simulink model "asbCubeSatArchModel"  (R2025b)
settings: configuration reference "CubeSatConfigSet" (kept outside this file)
InitFcn:
  | detectChangeOrbitalElements;
settings Model: DataDictionary=asbCubeSatArchInterfaceData.sldd  Creator=The MathWorks, Inc.  LastModifiedBy=The MathWorks, Inc.
settings ConfigSetRef: SourceName=CubeSatConfigSet

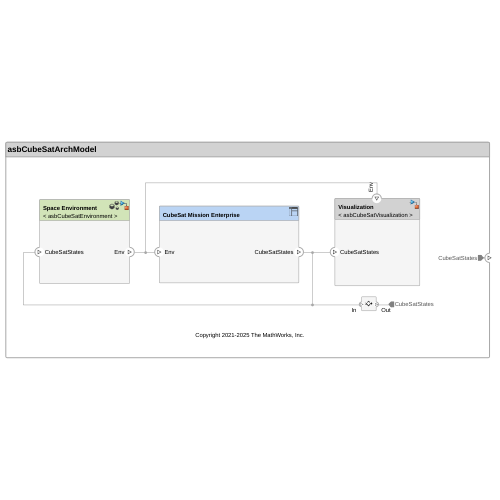
[thumbnail: Simulink's stored preview of the top-level diagram]
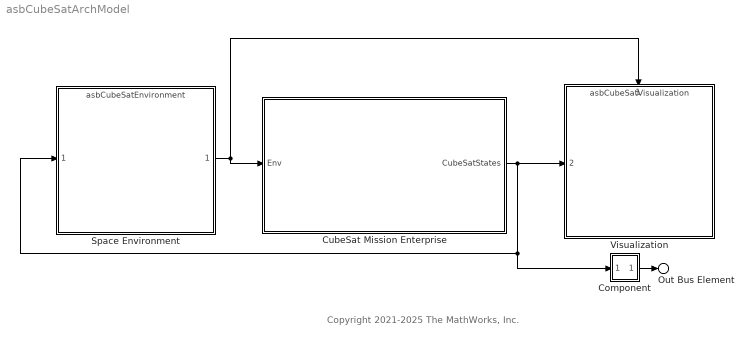
== system asbCubeSatArchModel ==
  note: Copyright 2021-2025 The MathWorks, Inc.
  Component : Subsystem
      settings: PortSchema="{\"entries\":[{\"content\":{\"margin\":10,\"minimumSpacing\":15,\"sides\":[{\"content\":{\"connectorIds\":[\"In1\"]},\"type\":\"ConnectorPlacement.EquallySpacedRectSide\",\"uuid\":\"9886ff7d-e976-4db1-93a5-6c4881d35d20\"},{\"content\":{\"connectorIds\":[\"Out1\"],\"side\":\"RIGHT\"},\"type\":\"ConnectorPlacement.EquallySpacedRectSide\",\"uuid\":\"ddfda7ac-6297-4455-a293-3eb8c5cedc24\"},{\"content\":{\"connectorIds\":[],\"side\":\"TOP\"},\"type\":\"ConnectorPlacement.EquallySpacedRectSide\",\"uuid\":\"53df18f4-c3f2-41e9-b086-6e9f9df8353a\"}]},\"type\":\"ConnectorPlacement.EquallySpacedConnector\",\"uuid\":\"ec2e31ee-cd1e-423f-b63c-a0e50b4897cf\"}],\"packageUris\":[\"http://schema.mathworks.com/mf0/Connector/R2020b\"],\"version\":\"1.0\"}"
  CubeSat Mission Enterprise : Subsystem  RequirementInfo="{}  %GIDa_b28b2482_6772_472c_87a3_7f97e1661d65"
      settings: PortSchema="{\"entries\":[{\"content\":{\"headerSize\":26,\"margin\":15,\"minimumSpacing\":25,\"sides\":[{\"content\":{\"connectorIds\":[\"In1\"]},\"type\":\"ConnectorPlacement.EquallySpacedRectSide\",\"uuid\":\"9b45e59d-ccd6-4576-99ba-beb2b78ee3b5\"},{\"content\":{\"connectorIds\":[\"Out1\"],\"side\":\"RIGHT\"},\"type\":\"ConnectorPlacement.EquallySpacedRectSide\",\"uuid\":\"e86d53dc-9e16-4af5-b392-fbf304437072\"},{\"content\":{\"connectorIds\":[],\"side\":\"TOP\"},\"type\":\"ConnectorPlacement.EquallySpacedRectSide\",\"uuid\":\"edfd08ba-6cd1-4548-8657-f8bd2c19a2e8\"}]},\"type\":\"ConnectorPlacement.EquallySpacedConnector\",\"uuid\":\"6ec86e3f-e232-4d2b-9702-b7c5151da82d\"}],\"packageUris\":[\"http://schema.mathworks.com/mf0/Connector/R2020b\"],\"version\":\"1.0\"}"
  Space Environment : ModelReference  ModelNameDialog=asbCubeSatEnvironment.slx  SimulationMode=Normal  ModelReferenceVersion=10.1
      settings: PortSchema="{\"entries\":[{\"content\":{\"headerSize\":38,\"margin\":15,\"minimumSpacing\":25,\"sides\":[{\"content\":{\"connectorIds\":[\"In1\"]},\"type\":\"ConnectorPlacement.EquallySpacedRectSide\",\"uuid\":\"f3e38669-0fba-438a-830e-4ecb3c477208\"},{\"content\":{\"connectorIds\":[\"Out1\"],\"side\":\"RIGHT\"},\"type\":\"ConnectorPlacement.EquallySpacedRectSide\",\"uuid\":\"56bbb7a2-868c-414d-930b-0bd7cd2045f0\"},{\"content\":{\"connectorIds\":[],\"side\":\"TOP\"},\"type\":\"ConnectorPlacement.EquallySpacedRectSide\",\"uuid\":\"88870cdb-fdfd-417b-9994-916f0d4ae524\"}]},\"type\":\"ConnectorPlacement.EquallySpacedConnector\",\"uuid\":\"741cde9d-e7e9-40ac-ba7b-7a3de3d6b210\"}],\"packageUris\":[\"http://schema.mathworks.com/mf0/Connector/19700101\"],\"version\":\"1.0\"}"
  Visualization : ModelReference  ModelNameDialog=asbCubeSatVisualization  SimulationMode=Normal  ModelReferenceVersion=11.7
      settings: PortSchema="{\"entries\":[{\"content\":{\"headerSize\":38,\"margin\":15,\"minimumSpacing\":25,\"sides\":[{\"content\":{\"connectorIds\":[\"In2\"]},\"type\":\"ConnectorPlacement.EquallySpacedRectSide\",\"uuid\":\"11899bdf-e452-4ab3-837e-0cb9b9384128\"},{\"content\":{\"connectorIds\":[],\"side\":\"RIGHT\"},\"type\":\"ConnectorPlacement.EquallySpacedRectSide\",\"uuid\":\"e13bda72-6c98-45bd-b419-0150b74f0acb\"},{\"content\":{\"connectorIds\":[\"In1\"],\"side\":\"TOP\"},\"type\":\"ConnectorPlacement.EquallySpacedRectSide\",\"uuid\":\"557a35da-b63d-4ba5-9926-82fbb2616f97\"}]},\"type\":\"ConnectorPlacement.EquallySpacedConnector\",\"uuid\":\"5fda5664-0755-42bb-a997-eaa89ad1d59d\"}],\"packageUris\":[\"http://schema.mathworks.com/mf0/Connector/R2020b\"],\"version\":\"1.0\"}"
  Out Bus Element : Outport  PortName=CubeSatStates
  wires:
  Space Environment/1 -> Visualization/1, CubeSat Mission Enterprise/1(Env)
  CubeSat Mission Enterprise/1(CubeSatStates) -> Component/1(In), Space Environment/1, Visualization/2
  Component/1(Out) -> Out Bus Element/1

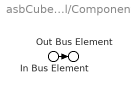
== system asbCubeSatArchModel/Component ==
  In Bus Element : Inport  PortName=In
  Out Bus Element : Outport  PortName=Out
  wires:
  In Bus Element/1 -> Out Bus Element/1

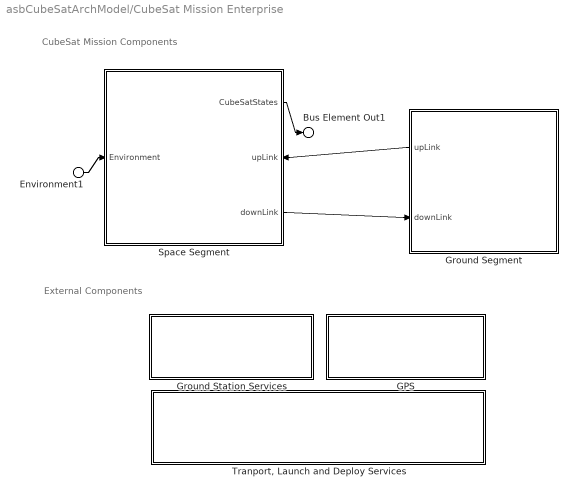
== system asbCubeSatArchModel/CubeSat Mission Enterprise ==
  note: CubeSat Mission Components
  note: External Components
  Environment1 : Inport  PortName=Env
  GPS : Subsystem
      settings: PortSchema="{\"entries\":[{\"content\":{\"headerSize\":26,\"margin\":15,\"minimumSpacing\":25,\"sides\":[{\"content\":{\"connectorIds\":[]},\"type\":\"ConnectorPlacement.EquallySpacedRectSide\",\"uuid\":\"9b45e59d-ccd6-4576-99ba-beb2b78ee3b5\"},{\"content\":{\"connectorIds\":[],\"side\":\"RIGHT\"},\"type\":\"ConnectorPlacement.EquallySpacedRectSide\",\"uuid\":\"e86d53dc-9e16-4af5-b392-fbf304437072\"},{\"content\":{\"connectorIds\":[],\"side\":\"TOP\"},\"type\":\"ConnectorPlacement.EquallySpacedRectSide\",\"uuid\":\"edfd08ba-6cd1-4548-8657-f8bd2c19a2e8\"}]},\"type\":\"ConnectorPlacement.EquallySpacedConnector\",\"uuid\":\"6ec86e3f-e232-4d2b-9702-b7c5151da82d\"}],\"packageUris\":[\"http://schema.mathworks.com/mf0/Connector/19700101\"],\"version\":\"1.0\"}"
  Ground Segment : Subsystem  RequirementInfo="{}  %GIDa_b06ae174_6660_44fc_ae78_7625ee106db0"
      settings: PortSchema="{\"entries\":[{\"content\":{\"headerSize\":26,\"margin\":15,\"minimumSpacing\":25,\"sides\":[{\"content\":{\"connectorIds\":[\"Out1\",\"In1\"]},\"type\":\"ConnectorPlacement.EquallySpacedRectSide\",\"uuid\":\"9b45e59d-ccd6-4576-99ba-beb2b78ee3b5\"},{\"content\":{\"connectorIds\":[],\"side\":\"RIGHT\"},\"type\":\"ConnectorPlacement.EquallySpacedRectSide\",\"uuid\":\"e86d53dc-9e16-4af5-b392-fbf304437072\"},{\"content\":{\"connectorIds\":[],\"side\":\"TOP\"},\"type\":\"ConnectorPlacement.EquallySpacedRectSide\",\"uuid\":\"edfd08ba-6cd1-4548-8657-f8bd2c19a2e8\"}]},\"type\":\"ConnectorPlacement.EquallySpacedConnector\",\"uuid\":\"6ec86e3f-e232-4d2b-9702-b7c5151da82d\"}],\"packageUris\":[\"http://schema.mathworks.com/mf0/Connector/19700101\"],\"version\":\"1.0\"}"
  Ground Station Services : Subsystem
      settings: PortSchema="{\"entries\":[{\"content\":{\"headerSize\":26,\"margin\":15,\"minimumSpacing\":25,\"sides\":[{\"content\":{\"connectorIds\":[]},\"type\":\"ConnectorPlacement.EquallySpacedRectSide\",\"uuid\":\"9b45e59d-ccd6-4576-99ba-beb2b78ee3b5\"},{\"content\":{\"connectorIds\":[],\"side\":\"RIGHT\"},\"type\":\"ConnectorPlacement.EquallySpacedRectSide\",\"uuid\":\"e86d53dc-9e16-4af5-b392-fbf304437072\"},{\"content\":{\"connectorIds\":[],\"side\":\"TOP\"},\"type\":\"ConnectorPlacement.EquallySpacedRectSide\",\"uuid\":\"edfd08ba-6cd1-4548-8657-f8bd2c19a2e8\"}]},\"type\":\"ConnectorPlacement.EquallySpacedConnector\",\"uuid\":\"6ec86e3f-e232-4d2b-9702-b7c5151da82d\"}],\"packageUris\":[\"http://schema.mathworks.com/mf0/Connector/19700101\"],\"version\":\"1.0\"}"
  Space Segment : Subsystem  RequirementInfo="{}  %GIDa_d5559e4d_919a_44dc_b881_614a5dae06b6"
      settings: PortSchema="{\"entries\":[{\"content\":{\"headerSize\":26,\"margin\":15,\"minimumSpacing\":25,\"sides\":[{\"content\":{\"connectorIds\":[\"In2\"]},\"type\":\"ConnectorPlacement.EquallySpacedRectSide\",\"uuid\":\"9b45e59d-ccd6-4576-99ba-beb2b78ee3b5\"},{\"content\":{\"connectorIds\":[\"Out1\",\"In1\",\"Out2\"],\"side\":\"RIGHT\"},\"type\":\"ConnectorPlacement.EquallySpacedRectSide\",\"uuid\":\"e86d53dc-9e16-4af5-b392-fbf304437072\"},{\"content\":{\"connectorIds\":[],\"side\":\"TOP\"},\"type\":\"ConnectorPlacement.EquallySpacedRectSide\",\"uuid\":\"edfd08ba-6cd1-4548-8657-f8bd2c19a2e8\"}]},\"type\":\"ConnectorPlacement.EquallySpacedConnector\",\"uuid\":\"6ec86e3f-e232-4d2b-9702-b7c5151da82d\"}],\"packageUris\":[\"http://schema.mathworks.com/mf0/Connector/R2020b\"],\"version\":\"1.0\"}"
  "Tranport, Launch and Deploy Services" : Subsystem
      settings: PortSchema="{\"entries\":[{\"content\":{\"headerSize\":26,\"margin\":15,\"minimumSpacing\":25,\"sides\":[{\"content\":{\"connectorIds\":[]},\"type\":\"ConnectorPlacement.EquallySpacedRectSide\",\"uuid\":\"9b45e59d-ccd6-4576-99ba-beb2b78ee3b5\"},{\"content\":{\"connectorIds\":[],\"side\":\"RIGHT\"},\"type\":\"ConnectorPlacement.EquallySpacedRectSide\",\"uuid\":\"e86d53dc-9e16-4af5-b392-fbf304437072\"},{\"content\":{\"connectorIds\":[],\"side\":\"TOP\"},\"type\":\"ConnectorPlacement.EquallySpacedRectSide\",\"uuid\":\"edfd08ba-6cd1-4548-8657-f8bd2c19a2e8\"}]},\"type\":\"ConnectorPlacement.EquallySpacedConnector\",\"uuid\":\"6ec86e3f-e232-4d2b-9702-b7c5151da82d\"}],\"packageUris\":[\"http://schema.mathworks.com/mf0/Connector/19700101\"],\"version\":\"1.0\"}"
  Bus Element Out1 : Outport  PortName=CubeSatStates
  wires:
  Environment1/1 -> Space Segment/2(Environment)
  Ground Segment/1(upLink) -> Space Segment/1(upLink)
  Space Segment/2(downLink) -> Ground Segment/1(downLink)
  Space Segment/1(CubeSatStates) -> Bus Element Out1/1

== system asbCubeSatArchModel/CubeSat Mission Enterprise/GPS ==

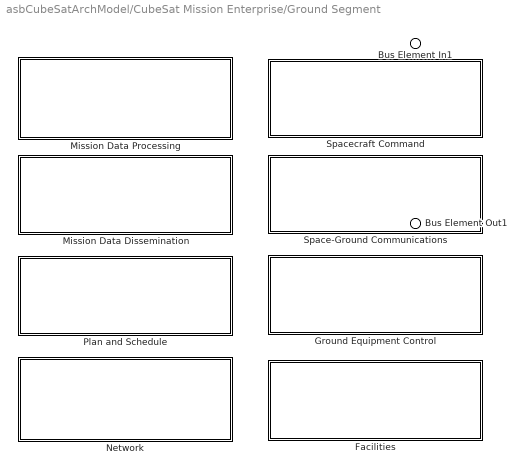
== system asbCubeSatArchModel/CubeSat Mission Enterprise/Ground Segment ==
  Bus Element In1 : Inport  PortName=downLink
  Facilities : Subsystem
      settings: PortSchema="{\"entries\":[{\"content\":{\"headerSize\":26,\"margin\":15,\"minimumSpacing\":25,\"sides\":[{\"content\":{\"connectorIds\":[]},\"type\":\"ConnectorPlacement.EquallySpacedRectSide\",\"uuid\":\"ec0b20de-43af-4595-9773-1ccab80dcb2a\"},{\"content\":{\"connectorIds\":[],\"side\":\"RIGHT\"},\"type\":\"ConnectorPlacement.EquallySpacedRectSide\",\"uuid\":\"ac6e6885-e3fb-4062-8a30-0baee43cecf2\"},{\"content\":{\"connectorIds\":[],\"side\":\"TOP\"},\"type\":\"ConnectorPlacement.EquallySpacedRectSide\",\"uuid\":\"2a1a79cc-6d5a-466f-8cc8-4618e952e6e8\"}]},\"type\":\"ConnectorPlacement.EquallySpacedConnector\",\"uuid\":\"4eb0413c-b7e8-4869-aa38-85b4ce7d1395\"}],\"packageUris\":[\"http://schema.mathworks.com/mf0/Connector/R2020b\"],\"version\":\"1.0\"}"
  Ground Equipment Control : Subsystem
      settings: PortSchema="{\"entries\":[{\"content\":{\"headerSize\":26,\"margin\":15,\"minimumSpacing\":25,\"sides\":[{\"content\":{\"connectorIds\":[]},\"type\":\"ConnectorPlacement.EquallySpacedRectSide\",\"uuid\":\"9b45e59d-ccd6-4576-99ba-beb2b78ee3b5\"},{\"content\":{\"connectorIds\":[],\"side\":\"RIGHT\"},\"type\":\"ConnectorPlacement.EquallySpacedRectSide\",\"uuid\":\"e86d53dc-9e16-4af5-b392-fbf304437072\"},{\"content\":{\"connectorIds\":[],\"side\":\"TOP\"},\"type\":\"ConnectorPlacement.EquallySpacedRectSide\",\"uuid\":\"edfd08ba-6cd1-4548-8657-f8bd2c19a2e8\"}]},\"type\":\"ConnectorPlacement.EquallySpacedConnector\",\"uuid\":\"6ec86e3f-e232-4d2b-9702-b7c5151da82d\"}],\"packageUris\":[\"http://schema.mathworks.com/mf0/Connector/19700101\"],\"version\":\"1.0\"}"
  Mission Data Dissemination : Subsystem
      settings: PortSchema="{\"entries\":[{\"content\":{\"headerSize\":26,\"margin\":15,\"minimumSpacing\":25,\"sides\":[{\"content\":{\"connectorIds\":[]},\"type\":\"ConnectorPlacement.EquallySpacedRectSide\",\"uuid\":\"9b45e59d-ccd6-4576-99ba-beb2b78ee3b5\"},{\"content\":{\"connectorIds\":[],\"side\":\"RIGHT\"},\"type\":\"ConnectorPlacement.EquallySpacedRectSide\",\"uuid\":\"e86d53dc-9e16-4af5-b392-fbf304437072\"},{\"content\":{\"connectorIds\":[],\"side\":\"TOP\"},\"type\":\"ConnectorPlacement.EquallySpacedRectSide\",\"uuid\":\"edfd08ba-6cd1-4548-8657-f8bd2c19a2e8\"}]},\"type\":\"ConnectorPlacement.EquallySpacedConnector\",\"uuid\":\"6ec86e3f-e232-4d2b-9702-b7c5151da82d\"}],\"packageUris\":[\"http://schema.mathworks.com/mf0/Connector/R2020b\"],\"version\":\"1.0\"}"
  Mission Data Processing : Subsystem
      settings: PortSchema="{\"entries\":[{\"content\":{\"headerSize\":26,\"margin\":15,\"minimumSpacing\":25,\"sides\":[{\"content\":{\"connectorIds\":[]},\"type\":\"ConnectorPlacement.EquallySpacedRectSide\",\"uuid\":\"9b45e59d-ccd6-4576-99ba-beb2b78ee3b5\"},{\"content\":{\"connectorIds\":[],\"side\":\"RIGHT\"},\"type\":\"ConnectorPlacement.EquallySpacedRectSide\",\"uuid\":\"e86d53dc-9e16-4af5-b392-fbf304437072\"},{\"content\":{\"connectorIds\":[],\"side\":\"TOP\"},\"type\":\"ConnectorPlacement.EquallySpacedRectSide\",\"uuid\":\"edfd08ba-6cd1-4548-8657-f8bd2c19a2e8\"}]},\"type\":\"ConnectorPlacement.EquallySpacedConnector\",\"uuid\":\"6ec86e3f-e232-4d2b-9702-b7c5151da82d\"}],\"packageUris\":[\"http://schema.mathworks.com/mf0/Connector/19700101\"],\"version\":\"1.0\"}"
  Network : Subsystem
      settings: PortSchema="{\"entries\":[{\"content\":{\"headerSize\":26,\"margin\":15,\"minimumSpacing\":25,\"sides\":[{\"content\":{\"connectorIds\":[]},\"type\":\"ConnectorPlacement.EquallySpacedRectSide\",\"uuid\":\"9b45e59d-ccd6-4576-99ba-beb2b78ee3b5\"},{\"content\":{\"connectorIds\":[],\"side\":\"RIGHT\"},\"type\":\"ConnectorPlacement.EquallySpacedRectSide\",\"uuid\":\"e86d53dc-9e16-4af5-b392-fbf304437072\"},{\"content\":{\"connectorIds\":[],\"side\":\"TOP\"},\"type\":\"ConnectorPlacement.EquallySpacedRectSide\",\"uuid\":\"edfd08ba-6cd1-4548-8657-f8bd2c19a2e8\"}]},\"type\":\"ConnectorPlacement.EquallySpacedConnector\",\"uuid\":\"6ec86e3f-e232-4d2b-9702-b7c5151da82d\"}],\"packageUris\":[\"http://schema.mathworks.com/mf0/Connector/19700101\"],\"version\":\"1.0\"}"
  Plan and Schedule : Subsystem
      settings: PortSchema="{\"entries\":[{\"content\":{\"headerSize\":26,\"margin\":15,\"minimumSpacing\":25,\"sides\":[{\"content\":{\"connectorIds\":[]},\"type\":\"ConnectorPlacement.EquallySpacedRectSide\",\"uuid\":\"9b45e59d-ccd6-4576-99ba-beb2b78ee3b5\"},{\"content\":{\"connectorIds\":[],\"side\":\"RIGHT\"},\"type\":\"ConnectorPlacement.EquallySpacedRectSide\",\"uuid\":\"e86d53dc-9e16-4af5-b392-fbf304437072\"},{\"content\":{\"connectorIds\":[],\"side\":\"TOP\"},\"type\":\"ConnectorPlacement.EquallySpacedRectSide\",\"uuid\":\"edfd08ba-6cd1-4548-8657-f8bd2c19a2e8\"}]},\"type\":\"ConnectorPlacement.EquallySpacedConnector\",\"uuid\":\"6ec86e3f-e232-4d2b-9702-b7c5151da82d\"}],\"packageUris\":[\"http://schema.mathworks.com/mf0/Connector/19700101\"],\"version\":\"1.0\"}"
  Space-Ground Communications : Subsystem
      settings: PortSchema="{\"entries\":[{\"content\":{\"headerSize\":26,\"margin\":15,\"minimumSpacing\":25,\"sides\":[{\"content\":{\"connectorIds\":[]},\"type\":\"ConnectorPlacement.EquallySpacedRectSide\",\"uuid\":\"9b45e59d-ccd6-4576-99ba-beb2b78ee3b5\"},{\"content\":{\"connectorIds\":[],\"side\":\"RIGHT\"},\"type\":\"ConnectorPlacement.EquallySpacedRectSide\",\"uuid\":\"e86d53dc-9e16-4af5-b392-fbf304437072\"},{\"content\":{\"connectorIds\":[],\"side\":\"TOP\"},\"type\":\"ConnectorPlacement.EquallySpacedRectSide\",\"uuid\":\"edfd08ba-6cd1-4548-8657-f8bd2c19a2e8\"}]},\"type\":\"ConnectorPlacement.EquallySpacedConnector\",\"uuid\":\"6ec86e3f-e232-4d2b-9702-b7c5151da82d\"}],\"packageUris\":[\"http://schema.mathworks.com/mf0/Connector/R2020b\"],\"version\":\"1.0\"}"
  Spacecraft Command : Subsystem
      settings: PortSchema="{\"entries\":[{\"content\":{\"headerSize\":26,\"margin\":15,\"minimumSpacing\":25,\"sides\":[{\"content\":{\"connectorIds\":[]},\"type\":\"ConnectorPlacement.EquallySpacedRectSide\",\"uuid\":\"9b45e59d-ccd6-4576-99ba-beb2b78ee3b5\"},{\"content\":{\"connectorIds\":[],\"side\":\"RIGHT\"},\"type\":\"ConnectorPlacement.EquallySpacedRectSide\",\"uuid\":\"e86d53dc-9e16-4af5-b392-fbf304437072\"},{\"content\":{\"connectorIds\":[],\"side\":\"TOP\"},\"type\":\"ConnectorPlacement.EquallySpacedRectSide\",\"uuid\":\"edfd08ba-6cd1-4548-8657-f8bd2c19a2e8\"}]},\"type\":\"ConnectorPlacement.EquallySpacedConnector\",\"uuid\":\"6ec86e3f-e232-4d2b-9702-b7c5151da82d\"}],\"packageUris\":[\"http://schema.mathworks.com/mf0/Connector/R2020b\"],\"version\":\"1.0\"}"
  Bus Element Out1 : Outport  PortName=upLink

== system asbCubeSatArchModel/CubeSat Mission Enterprise/Ground Station Services ==

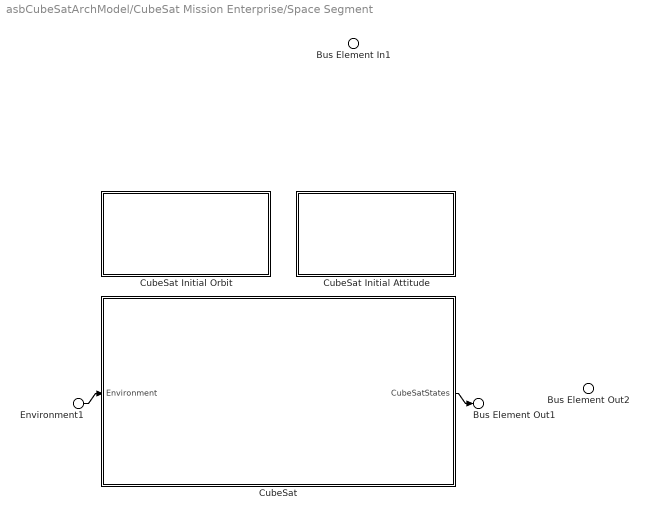
== system asbCubeSatArchModel/CubeSat Mission Enterprise/Space Segment ==
  Bus Element In1 : Inport  PortName=upLink
  Environment1 : Inport  Port=2  PortName=Environment
  CubeSat : Subsystem
      settings: PortSchema="{\"entries\":[{\"content\":{\"headerSize\":26,\"margin\":15,\"minimumSpacing\":25,\"sides\":[{\"content\":{\"connectorIds\":[\"In1\"]},\"type\":\"ConnectorPlacement.EquallySpacedRectSide\",\"uuid\":\"9b45e59d-ccd6-4576-99ba-beb2b78ee3b5\"},{\"content\":{\"connectorIds\":[\"Out1\"],\"side\":\"RIGHT\"},\"type\":\"ConnectorPlacement.EquallySpacedRectSide\",\"uuid\":\"e86d53dc-9e16-4af5-b392-fbf304437072\"},{\"content\":{\"connectorIds\":[],\"side\":\"TOP\"},\"type\":\"ConnectorPlacement.EquallySpacedRectSide\",\"uuid\":\"edfd08ba-6cd1-4548-8657-f8bd2c19a2e8\"}]},\"type\":\"ConnectorPlacement.EquallySpacedConnector\",\"uuid\":\"6ec86e3f-e232-4d2b-9702-b7c5151da82d\"}],\"packageUris\":[\"http://schema.mathworks.com/mf0/Connector/R2020b\"],\"version\":\"1.0\"}"
  CubeSat Initial Attitude : Subsystem
      settings: PortSchema="{\"entries\":[{\"content\":{\"headerSize\":26,\"margin\":15,\"minimumSpacing\":25,\"sides\":[{\"content\":{\"connectorIds\":[]},\"type\":\"ConnectorPlacement.EquallySpacedRectSide\",\"uuid\":\"9b45e59d-ccd6-4576-99ba-beb2b78ee3b5\"},{\"content\":{\"connectorIds\":[],\"side\":\"RIGHT\"},\"type\":\"ConnectorPlacement.EquallySpacedRectSide\",\"uuid\":\"e86d53dc-9e16-4af5-b392-fbf304437072\"},{\"content\":{\"connectorIds\":[],\"side\":\"TOP\"},\"type\":\"ConnectorPlacement.EquallySpacedRectSide\",\"uuid\":\"edfd08ba-6cd1-4548-8657-f8bd2c19a2e8\"}]},\"type\":\"ConnectorPlacement.EquallySpacedConnector\",\"uuid\":\"6ec86e3f-e232-4d2b-9702-b7c5151da82d\"}],\"packageUris\":[\"http://schema.mathworks.com/mf0/Connector/R2020b\"],\"version\":\"1.0\"}"
  CubeSat Initial Orbit : Subsystem  RequirementInfo="{}  %GIDa_6b67bace_5f11_42a0_bcc1_193026a664c1"
      settings: PortSchema="{\"entries\":[{\"content\":{\"headerSize\":26,\"margin\":15,\"minimumSpacing\":25,\"sides\":[{\"content\":{\"connectorIds\":[]},\"type\":\"ConnectorPlacement.EquallySpacedRectSide\",\"uuid\":\"9b45e59d-ccd6-4576-99ba-beb2b78ee3b5\"},{\"content\":{\"connectorIds\":[],\"side\":\"RIGHT\"},\"type\":\"ConnectorPlacement.EquallySpacedRectSide\",\"uuid\":\"e86d53dc-9e16-4af5-b392-fbf304437072\"},{\"content\":{\"connectorIds\":[],\"side\":\"TOP\"},\"type\":\"ConnectorPlacement.EquallySpacedRectSide\",\"uuid\":\"edfd08ba-6cd1-4548-8657-f8bd2c19a2e8\"}]},\"type\":\"ConnectorPlacement.EquallySpacedConnector\",\"uuid\":\"6ec86e3f-e232-4d2b-9702-b7c5151da82d\"}],\"packageUris\":[\"http://schema.mathworks.com/mf0/Connector/R2020b\"],\"version\":\"1.0\"}"
  Bus Element Out1 : Outport  PortName=CubeSatStates
  Bus Element Out2 : Outport  Port=2  PortName=downLink
  wires:
  Environment1/1 -> CubeSat/1(Environment)
  CubeSat/1(CubeSatStates) -> Bus Element Out1/1

== system asbCubeSatArchModel/CubeSat Mission Enterprise/Tranport, Launch and Deploy Services ==

== system asbCubeSatArchModel/CubeSat Mission Enterprise/Ground Segment/Facilities ==

== system asbCubeSatArchModel/CubeSat Mission Enterprise/Ground Segment/Ground Equipment Control ==

== system asbCubeSatArchModel/CubeSat Mission Enterprise/Ground Segment/Mission Data Dissemination ==

== system asbCubeSatArchModel/CubeSat Mission Enterprise/Ground Segment/Mission Data Processing ==

== system asbCubeSatArchModel/CubeSat Mission Enterprise/Ground Segment/Network ==

== system asbCubeSatArchModel/CubeSat Mission Enterprise/Ground Segment/Plan and Schedule ==

== system asbCubeSatArchModel/CubeSat Mission Enterprise/Ground Segment/Space-Ground Communications ==

== system asbCubeSatArchModel/CubeSat Mission Enterprise/Ground Segment/Spacecraft Command ==

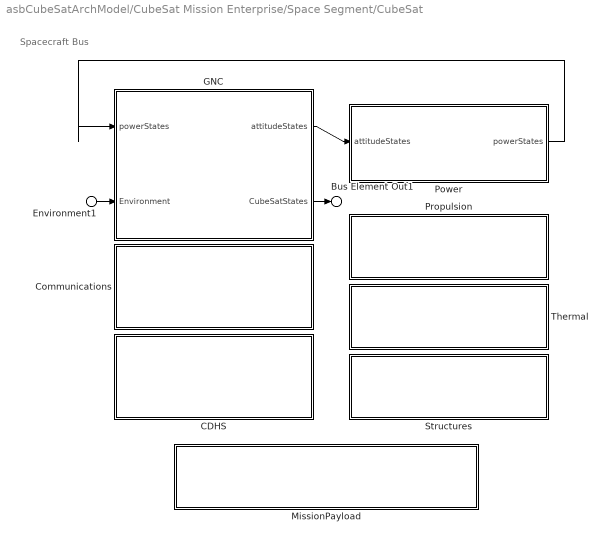
== system asbCubeSatArchModel/CubeSat Mission Enterprise/Space Segment/CubeSat ==
  note: Spacecraft Bus
  Environment1 : Inport  PortName=Environment
  CDHS : Subsystem
      settings: PortSchema="{\"entries\":[{\"content\":{\"headerSize\":26,\"margin\":15,\"minimumSpacing\":25,\"sides\":[{\"content\":{\"connectorIds\":[]},\"type\":\"ConnectorPlacement.EquallySpacedRectSide\",\"uuid\":\"9b45e59d-ccd6-4576-99ba-beb2b78ee3b5\"},{\"content\":{\"connectorIds\":[],\"side\":\"RIGHT\"},\"type\":\"ConnectorPlacement.EquallySpacedRectSide\",\"uuid\":\"e86d53dc-9e16-4af5-b392-fbf304437072\"},{\"content\":{\"connectorIds\":[],\"side\":\"TOP\"},\"type\":\"ConnectorPlacement.EquallySpacedRectSide\",\"uuid\":\"edfd08ba-6cd1-4548-8657-f8bd2c19a2e8\"}]},\"type\":\"ConnectorPlacement.EquallySpacedConnector\",\"uuid\":\"6ec86e3f-e232-4d2b-9702-b7c5151da82d\"}],\"packageUris\":[\"http://schema.mathworks.com/mf0/Connector/19700101\"],\"version\":\"1.0\"}"
  Communications : Subsystem
      settings: PortSchema="{\"entries\":[{\"content\":{\"headerSize\":26,\"margin\":15,\"minimumSpacing\":25,\"sides\":[{\"content\":{\"connectorIds\":[]},\"type\":\"ConnectorPlacement.EquallySpacedRectSide\",\"uuid\":\"9b45e59d-ccd6-4576-99ba-beb2b78ee3b5\"},{\"content\":{\"connectorIds\":[],\"side\":\"RIGHT\"},\"type\":\"ConnectorPlacement.EquallySpacedRectSide\",\"uuid\":\"e86d53dc-9e16-4af5-b392-fbf304437072\"},{\"content\":{\"connectorIds\":[],\"side\":\"TOP\"},\"type\":\"ConnectorPlacement.EquallySpacedRectSide\",\"uuid\":\"edfd08ba-6cd1-4548-8657-f8bd2c19a2e8\"}]},\"type\":\"ConnectorPlacement.EquallySpacedConnector\",\"uuid\":\"6ec86e3f-e232-4d2b-9702-b7c5151da82d\"}],\"packageUris\":[\"http://schema.mathworks.com/mf0/Connector/19700101\"],\"version\":\"1.0\"}"
  GNC : Subsystem  RequirementInfo="{}  %GIDa_dce94860_2c89_4024_b166_6039f795e48e"
      settings: PortSchema="{\"entries\":[{\"content\":{\"headerSize\":26,\"margin\":15,\"minimumSpacing\":25,\"sides\":[{\"content\":{\"connectorIds\":[\"In1\",\"In2\"]},\"type\":\"ConnectorPlacement.EquallySpacedRectSide\",\"uuid\":\"9b45e59d-ccd6-4576-99ba-beb2b78ee3b5\"},{\"content\":{\"connectorIds\":[\"Out1\",\"Out2\"],\"side\":\"RIGHT\"},\"type\":\"ConnectorPlacement.EquallySpacedRectSide\",\"uuid\":\"e86d53dc-9e16-4af5-b392-fbf304437072\"},{\"content\":{\"connectorIds\":[],\"side\":\"TOP\"},\"type\":\"ConnectorPlacement.EquallySpacedRectSide\",\"uuid\":\"edfd08ba-6cd1-4548-8657-f8bd2c19a2e8\"}]},\"type\":\"ConnectorPlacement.EquallySpacedConnector\",\"uuid\":\"6ec86e3f-e232-4d2b-9702-b7c5151da82d\"}],\"packageUris\":[\"http://schema.mathworks.com/mf0/Connector/R2020b\"],\"version\":\"1.0\"}"
  MissionPayload : Subsystem
      settings: PortSchema="{\"entries\":[{\"content\":{\"headerSize\":26,\"margin\":15,\"minimumSpacing\":25,\"sides\":[{\"content\":{\"connectorIds\":[]},\"type\":\"ConnectorPlacement.EquallySpacedRectSide\",\"uuid\":\"9b45e59d-ccd6-4576-99ba-beb2b78ee3b5\"},{\"content\":{\"connectorIds\":[],\"side\":\"RIGHT\"},\"type\":\"ConnectorPlacement.EquallySpacedRectSide\",\"uuid\":\"e86d53dc-9e16-4af5-b392-fbf304437072\"},{\"content\":{\"connectorIds\":[],\"side\":\"TOP\"},\"type\":\"ConnectorPlacement.EquallySpacedRectSide\",\"uuid\":\"edfd08ba-6cd1-4548-8657-f8bd2c19a2e8\"}]},\"type\":\"ConnectorPlacement.EquallySpacedConnector\",\"uuid\":\"6ec86e3f-e232-4d2b-9702-b7c5151da82d\"}],\"packageUris\":[\"http://schema.mathworks.com/mf0/Connector/R2020b\"],\"version\":\"1.0\"}"
  Power : Subsystem
      settings: PortSchema="{\"entries\":[{\"content\":{\"headerSize\":26,\"margin\":15,\"minimumSpacing\":25,\"sides\":[{\"content\":{\"connectorIds\":[\"In1\"]},\"type\":\"ConnectorPlacement.EquallySpacedRectSide\",\"uuid\":\"9b45e59d-ccd6-4576-99ba-beb2b78ee3b5\"},{\"content\":{\"connectorIds\":[\"Out1\"],\"side\":\"RIGHT\"},\"type\":\"ConnectorPlacement.EquallySpacedRectSide\",\"uuid\":\"e86d53dc-9e16-4af5-b392-fbf304437072\"},{\"content\":{\"connectorIds\":[],\"side\":\"TOP\"},\"type\":\"ConnectorPlacement.EquallySpacedRectSide\",\"uuid\":\"edfd08ba-6cd1-4548-8657-f8bd2c19a2e8\"}]},\"type\":\"ConnectorPlacement.EquallySpacedConnector\",\"uuid\":\"6ec86e3f-e232-4d2b-9702-b7c5151da82d\"}],\"packageUris\":[\"http://schema.mathworks.com/mf0/Connector/19700101\"],\"version\":\"1.0\"}"
  Propulsion : Subsystem
      settings: PortSchema="{\"entries\":[{\"content\":{\"headerSize\":26,\"margin\":15,\"minimumSpacing\":25,\"sides\":[{\"content\":{\"connectorIds\":[]},\"type\":\"ConnectorPlacement.EquallySpacedRectSide\",\"uuid\":\"9b45e59d-ccd6-4576-99ba-beb2b78ee3b5\"},{\"content\":{\"connectorIds\":[],\"side\":\"RIGHT\"},\"type\":\"ConnectorPlacement.EquallySpacedRectSide\",\"uuid\":\"e86d53dc-9e16-4af5-b392-fbf304437072\"},{\"content\":{\"connectorIds\":[],\"side\":\"TOP\"},\"type\":\"ConnectorPlacement.EquallySpacedRectSide\",\"uuid\":\"edfd08ba-6cd1-4548-8657-f8bd2c19a2e8\"}]},\"type\":\"ConnectorPlacement.EquallySpacedConnector\",\"uuid\":\"6ec86e3f-e232-4d2b-9702-b7c5151da82d\"}],\"packageUris\":[\"http://schema.mathworks.com/mf0/Connector/R2020b\"],\"version\":\"1.0\"}"
  Structures : Subsystem
      settings: PortSchema="{\"entries\":[{\"content\":{\"headerSize\":26,\"margin\":15,\"minimumSpacing\":25,\"sides\":[{\"content\":{\"connectorIds\":[]},\"type\":\"ConnectorPlacement.EquallySpacedRectSide\",\"uuid\":\"9b45e59d-ccd6-4576-99ba-beb2b78ee3b5\"},{\"content\":{\"connectorIds\":[],\"side\":\"RIGHT\"},\"type\":\"ConnectorPlacement.EquallySpacedRectSide\",\"uuid\":\"e86d53dc-9e16-4af5-b392-fbf304437072\"},{\"content\":{\"connectorIds\":[],\"side\":\"TOP\"},\"type\":\"ConnectorPlacement.EquallySpacedRectSide\",\"uuid\":\"edfd08ba-6cd1-4548-8657-f8bd2c19a2e8\"}]},\"type\":\"ConnectorPlacement.EquallySpacedConnector\",\"uuid\":\"6ec86e3f-e232-4d2b-9702-b7c5151da82d\"}],\"packageUris\":[\"http://schema.mathworks.com/mf0/Connector/19700101\"],\"version\":\"1.0\"}"
  Thermal : Subsystem
      settings: PortSchema="{\"entries\":[{\"content\":{\"headerSize\":26,\"margin\":15,\"minimumSpacing\":25,\"sides\":[{\"content\":{\"connectorIds\":[]},\"type\":\"ConnectorPlacement.EquallySpacedRectSide\",\"uuid\":\"9b45e59d-ccd6-4576-99ba-beb2b78ee3b5\"},{\"content\":{\"connectorIds\":[],\"side\":\"RIGHT\"},\"type\":\"ConnectorPlacement.EquallySpacedRectSide\",\"uuid\":\"e86d53dc-9e16-4af5-b392-fbf304437072\"},{\"content\":{\"connectorIds\":[],\"side\":\"TOP\"},\"type\":\"ConnectorPlacement.EquallySpacedRectSide\",\"uuid\":\"edfd08ba-6cd1-4548-8657-f8bd2c19a2e8\"}]},\"type\":\"ConnectorPlacement.EquallySpacedConnector\",\"uuid\":\"6ec86e3f-e232-4d2b-9702-b7c5151da82d\"}],\"packageUris\":[\"http://schema.mathworks.com/mf0/Connector/R2020b\"],\"version\":\"1.0\"}"
  Bus Element Out1 : Outport  PortName=CubeSatStates
  wires:
  Environment1/1 -> GNC/2(Environment)
  GNC/1(attitudeStates) -> Power/1(attitudeStates)
  Power/1(powerStates) -> GNC/1(powerStates)
  GNC/2(CubeSatStates) -> Bus Element Out1/1

== system asbCubeSatArchModel/CubeSat Mission Enterprise/Space Segment/CubeSat Initial Attitude ==
  note: Use Attitude stereotype to set initial attitude state

== system asbCubeSatArchModel/CubeSat Mission Enterprise/Space Segment/CubeSat Initial Orbit ==
  note: Use Orbit stereotype to set initial orbit state

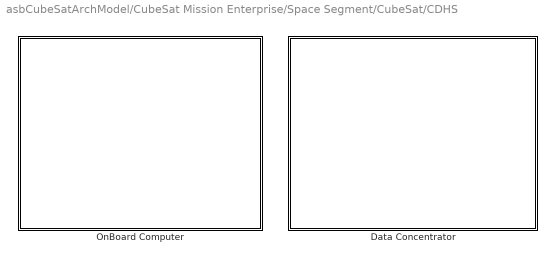
== system asbCubeSatArchModel/CubeSat Mission Enterprise/Space Segment/CubeSat/CDHS ==
  Data Concentrator : Subsystem
      settings: PortSchema="{\"entries\":[{\"content\":{\"headerSize\":26,\"margin\":15,\"minimumSpacing\":25,\"sides\":[{\"content\":{\"connectorIds\":[]},\"type\":\"ConnectorPlacement.EquallySpacedRectSide\",\"uuid\":\"5f91b340-2dca-474f-99b1-4cfb93e98d8a\"},{\"content\":{\"connectorIds\":[],\"side\":\"RIGHT\"},\"type\":\"ConnectorPlacement.EquallySpacedRectSide\",\"uuid\":\"d2e4d2f7-eaea-406c-8999-5255faa209a3\"},{\"content\":{\"connectorIds\":[],\"side\":\"TOP\"},\"type\":\"ConnectorPlacement.EquallySpacedRectSide\",\"uuid\":\"8064b484-3a4f-43f4-8560-07d3e2dea7d6\"}]},\"type\":\"ConnectorPlacement.EquallySpacedConnector\",\"uuid\":\"b547807e-0571-4405-b6f1-7ad363b80218\"}],\"packageUris\":[\"http://schema.mathworks.com/mf0/Connector/R2020b\"],\"version\":\"1.0\"}"
  OnBoard Computer : Subsystem
      settings: PortSchema="{\"entries\":[{\"content\":{\"headerSize\":26,\"margin\":15,\"minimumSpacing\":25,\"sides\":[{\"content\":{\"connectorIds\":[]},\"type\":\"ConnectorPlacement.EquallySpacedRectSide\",\"uuid\":\"5f91b340-2dca-474f-99b1-4cfb93e98d8a\"},{\"content\":{\"connectorIds\":[],\"side\":\"RIGHT\"},\"type\":\"ConnectorPlacement.EquallySpacedRectSide\",\"uuid\":\"d2e4d2f7-eaea-406c-8999-5255faa209a3\"},{\"content\":{\"connectorIds\":[],\"side\":\"TOP\"},\"type\":\"ConnectorPlacement.EquallySpacedRectSide\",\"uuid\":\"8064b484-3a4f-43f4-8560-07d3e2dea7d6\"}]},\"type\":\"ConnectorPlacement.EquallySpacedConnector\",\"uuid\":\"b547807e-0571-4405-b6f1-7ad363b80218\"}],\"packageUris\":[\"http://schema.mathworks.com/mf0/Connector/R2020b\"],\"version\":\"1.0\"}"

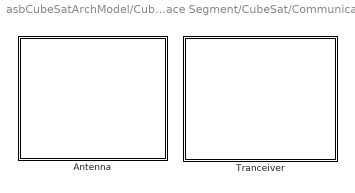
== system asbCubeSatArchModel/CubeSat Mission Enterprise/Space Segment/CubeSat/Communications ==
  Antenna : Subsystem
      settings: PortSchema="{\"entries\":[{\"content\":{\"headerSize\":26,\"margin\":15,\"minimumSpacing\":25,\"sides\":[{\"content\":{\"connectorIds\":[]},\"type\":\"ConnectorPlacement.EquallySpacedRectSide\",\"uuid\":\"5f91b340-2dca-474f-99b1-4cfb93e98d8a\"},{\"content\":{\"connectorIds\":[],\"side\":\"RIGHT\"},\"type\":\"ConnectorPlacement.EquallySpacedRectSide\",\"uuid\":\"d2e4d2f7-eaea-406c-8999-5255faa209a3\"},{\"content\":{\"connectorIds\":[],\"side\":\"TOP\"},\"type\":\"ConnectorPlacement.EquallySpacedRectSide\",\"uuid\":\"8064b484-3a4f-43f4-8560-07d3e2dea7d6\"}]},\"type\":\"ConnectorPlacement.EquallySpacedConnector\",\"uuid\":\"b547807e-0571-4405-b6f1-7ad363b80218\"}],\"packageUris\":[\"http://schema.mathworks.com/mf0/Connector/R2020b\"],\"version\":\"1.0\"}"
  Tranceiver : Subsystem
      settings: PortSchema="{\"entries\":[{\"content\":{\"headerSize\":26,\"margin\":15,\"minimumSpacing\":25,\"sides\":[{\"content\":{\"connectorIds\":[]},\"type\":\"ConnectorPlacement.EquallySpacedRectSide\",\"uuid\":\"5f91b340-2dca-474f-99b1-4cfb93e98d8a\"},{\"content\":{\"connectorIds\":[],\"side\":\"RIGHT\"},\"type\":\"ConnectorPlacement.EquallySpacedRectSide\",\"uuid\":\"d2e4d2f7-eaea-406c-8999-5255faa209a3\"},{\"content\":{\"connectorIds\":[],\"side\":\"TOP\"},\"type\":\"ConnectorPlacement.EquallySpacedRectSide\",\"uuid\":\"8064b484-3a4f-43f4-8560-07d3e2dea7d6\"}]},\"type\":\"ConnectorPlacement.EquallySpacedConnector\",\"uuid\":\"b547807e-0571-4405-b6f1-7ad363b80218\"}],\"packageUris\":[\"http://schema.mathworks.com/mf0/Connector/R2020b\"],\"version\":\"1.0\"}"

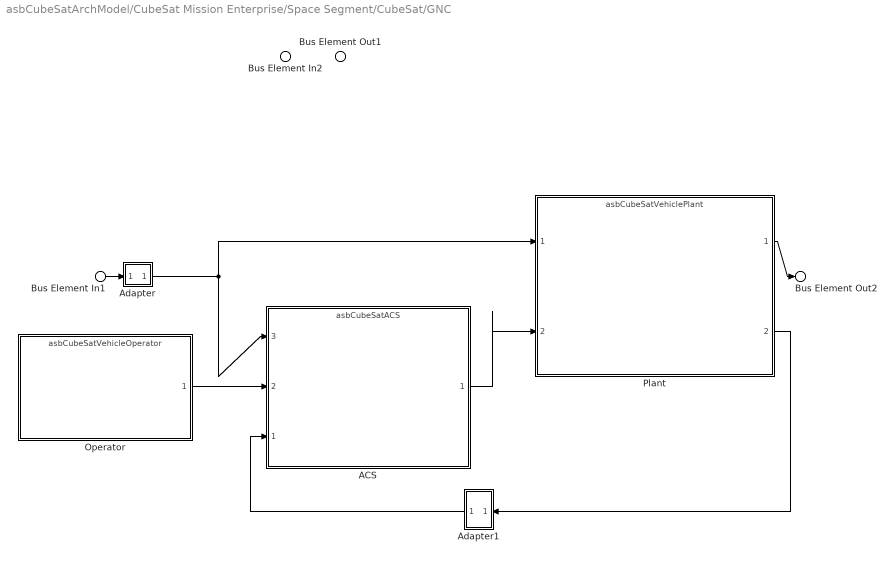
== system asbCubeSatArchModel/CubeSat Mission Enterprise/Space Segment/CubeSat/GNC ==
  Bus Element In2 : Inport  PortName=powerStates
  Bus Element In1 : Inport  Port=2  PortName=Environment
  ACS : ModelReference  ModelNameDialog=asbCubeSatACS  SimulationMode=Normal  ModelReferenceVersion=7.0
      settings: PortSchema="{\"entries\":[{\"content\":{\"headerSize\":38,\"margin\":15,\"minimumSpacing\":25,\"sides\":[{\"content\":{\"connectorIds\":[\"In3\",\"In2\",\"In1\"]},\"type\":\"ConnectorPlacement.EquallySpacedRectSide\",\"uuid\":\"0f167fc6-742e-49a6-ba84-7432b698566b\"},{\"content\":{\"connectorIds\":[\"Out1\"],\"side\":\"RIGHT\"},\"type\":\"ConnectorPlacement.EquallySpacedRectSide\",\"uuid\":\"3739c3b1-9e94-48d6-b273-772045adf57e\"},{\"content\":{\"connectorIds\":[],\"side\":\"TOP\"},\"type\":\"ConnectorPlacement.EquallySpacedRectSide\",\"uuid\":\"85e3313f-7b52-412d-a268-8976d9c4c82a\"},{\"content\":{\"connectorIds\":[],\"side\":\"HIDDEN\"},\"type\":\"ConnectorPlacement.EquallySpacedRectSide\",\"uuid\":\"31b4754e-d861-4dca-8700-99ce83c843d7\"}]},\"type\":\"ConnectorPlacement.EquallySpacedConnector\",\"uuid\":\"359d3eed-f1ba-4819-bbac-059d00dff13f\"}],\"packageUris\":[\"http://schema.mathworks.com/mf0/Connector/R2020b\"],\"version\":\"1.0\"}"
  Adapter : Subsystem
      settings: PortSchema="{\"entries\":[{\"content\":{\"margin\":10,\"minimumSpacing\":15,\"sides\":[{\"content\":{\"connectorIds\":[\"In1\"]},\"type\":\"ConnectorPlacement.EquallySpacedRectSide\",\"uuid\":\"0f167fc6-742e-49a6-ba84-7432b698566b\"},{\"content\":{\"connectorIds\":[\"Out1\"],\"side\":\"RIGHT\"},\"type\":\"ConnectorPlacement.EquallySpacedRectSide\",\"uuid\":\"3739c3b1-9e94-48d6-b273-772045adf57e\"},{\"content\":{\"connectorIds\":[],\"side\":\"TOP\"},\"type\":\"ConnectorPlacement.EquallySpacedRectSide\",\"uuid\":\"85e3313f-7b52-412d-a268-8976d9c4c82a\"},{\"content\":{\"connectorIds\":[],\"side\":\"HIDDEN\"},\"type\":\"ConnectorPlacement.EquallySpacedRectSide\",\"uuid\":\"31b4754e-d861-4dca-8700-99ce83c843d7\"}]},\"type\":\"ConnectorPlacement.EquallySpacedConnector\",\"uuid\":\"359d3eed-f1ba-4819-bbac-059d00dff13f\"}],\"packageUris\":[\"http://schema.mathworks.com/mf0/Connector/R2020b\"],\"version\":\"1.0\"}"
  Adapter1 : Subsystem
      settings: PortSchema="{\"entries\":[{\"content\":{\"margin\":10,\"minimumSpacing\":15,\"sides\":[{\"content\":{\"connectorIds\":[\"Out1\"]},\"type\":\"ConnectorPlacement.EquallySpacedRectSide\",\"uuid\":\"0f167fc6-742e-49a6-ba84-7432b698566b\"},{\"content\":{\"connectorIds\":[\"In1\"],\"side\":\"RIGHT\"},\"type\":\"ConnectorPlacement.EquallySpacedRectSide\",\"uuid\":\"3739c3b1-9e94-48d6-b273-772045adf57e\"},{\"content\":{\"connectorIds\":[],\"side\":\"TOP\"},\"type\":\"ConnectorPlacement.EquallySpacedRectSide\",\"uuid\":\"85e3313f-7b52-412d-a268-8976d9c4c82a\"},{\"content\":{\"connectorIds\":[],\"side\":\"HIDDEN\"},\"type\":\"ConnectorPlacement.EquallySpacedRectSide\",\"uuid\":\"31b4754e-d861-4dca-8700-99ce83c843d7\"}]},\"type\":\"ConnectorPlacement.EquallySpacedConnector\",\"uuid\":\"359d3eed-f1ba-4819-bbac-059d00dff13f\"}],\"packageUris\":[\"http://schema.mathworks.com/mf0/Connector/R2020b\"],\"version\":\"1.0\"}"
  Operator : ModelReference  ModelNameDialog=asbCubeSatVehicleOperator.slx  SimulationMode=Normal  ModelReferenceVersion=5.0
      settings: PortSchema="{\"entries\":[{\"content\":{\"headerSize\":38,\"margin\":15,\"minimumSpacing\":25,\"sides\":[{\"content\":{\"connectorIds\":[]},\"type\":\"ConnectorPlacement.EquallySpacedRectSide\",\"uuid\":\"0cfa3760-6acd-4ee9-b963-b5fbd04f8f00\"},{\"content\":{\"connectorIds\":[\"Out1\"],\"side\":\"RIGHT\"},\"type\":\"ConnectorPlacement.EquallySpacedRectSide\",\"uuid\":\"77ddd3d4-6692-4839-8cf9-45c7d2a217c2\"},{\"content\":{\"connectorIds\":[],\"side\":\"TOP\"},\"type\":\"ConnectorPlacement.EquallySpacedRectSide\",\"uuid\":\"8d936f89-fcb3-43a7-b6aa-fe007208be1f\"},{\"content\":{\"connectorIds\":[],\"side\":\"HIDDEN\"},\"type\":\"ConnectorPlacement.EquallySpacedRectSide\",\"uuid\":\"226e0ead-de34-4bf0-af80-010c29a26ac8\"}]},\"type\":\"ConnectorPlacement.EquallySpacedConnector\",\"uuid\":\"8760ac77-0d6c-4b36-b848-bf5fd4811ef2\"}],\"packageUris\":[\"http://schema.mathworks.com/mf0/Connector/R2020b\"],\"version\":\"1.0\"}"
  Plant : ModelReference  ModelNameDialog=asbCubeSatVehiclePlant.slx  SimulationMode=Normal  ModelReferenceVersion=6.0
      settings: PortSchema="{\"entries\":[{\"content\":{\"headerSize\":38,\"margin\":15,\"minimumSpacing\":25,\"sides\":[{\"content\":{\"connectorIds\":[\"In1\",\"In2\"]},\"type\":\"ConnectorPlacement.EquallySpacedRectSide\",\"uuid\":\"03f9f3cf-bad9-4ee2-9ea8-9738e2c4045a\"},{\"content\":{\"connectorIds\":[\"Out1\",\"Out2\"],\"side\":\"RIGHT\"},\"type\":\"ConnectorPlacement.EquallySpacedRectSide\",\"uuid\":\"a92bb464-fb2e-4a9d-9894-a6e38f24e9d5\"},{\"content\":{\"connectorIds\":[],\"side\":\"TOP\"},\"type\":\"ConnectorPlacement.EquallySpacedRectSide\",\"uuid\":\"549ebd3b-d1ab-424b-a511-2a627dad6dc4\"}]},\"type\":\"ConnectorPlacement.EquallySpacedConnector\",\"uuid\":\"0d138b15-5b32-4458-951b-b6abbba02272\"}],\"packageUris\":[\"http://schema.mathworks.com/mf0/Connector/R2020b\"],\"version\":\"1.0\"}"
  Bus Element Out1 : Outport  PortName=attitudeStates
  Bus Element Out2 : Outport  Port=2  PortName=CubeSatStates
  wires:
  Bus Element In1/1 -> Adapter/1(Environment)
  Adapter/1(Out) -> Plant/1, ACS/3
  ACS/1 -> Plant/2
  Plant/2 -> Adapter1/1(SensorsOut)
  Adapter1/1(Input) -> ACS/1
  Operator/1 -> ACS/2
  Plant/1 -> Bus Element Out2/1

== system asbCubeSatArchModel/CubeSat Mission Enterprise/Space Segment/CubeSat/MissionPayload ==

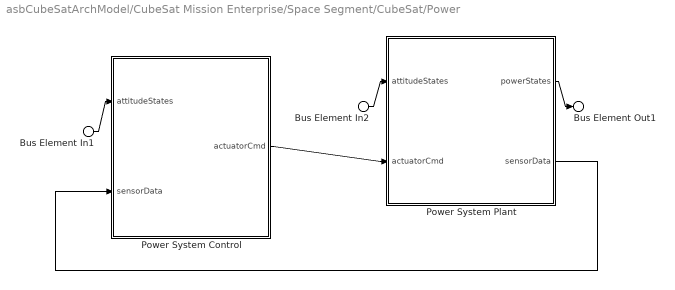
== system asbCubeSatArchModel/CubeSat Mission Enterprise/Space Segment/CubeSat/Power ==
  Bus Element In1 : Inport  PortName=attitudeStates
  Bus Element In2 : Inport  PortName=attitudeStates
  Power System Control : Subsystem  VariantControl=Choice_1
      settings: PortSchema="{\"entries\":[{\"content\":{\"headerSize\":26,\"margin\":15,\"minimumSpacing\":25,\"sides\":[{\"content\":{\"connectorIds\":[\"In1\",\"In2\"]},\"type\":\"ConnectorPlacement.EquallySpacedRectSide\",\"uuid\":\"796081c6-2161-46d9-94c7-9250e1efb39a\"},{\"content\":{\"connectorIds\":[\"Out1\"],\"side\":\"RIGHT\"},\"type\":\"ConnectorPlacement.EquallySpacedRectSide\",\"uuid\":\"b842dbfb-bf0a-4727-8e1c-eb47e2e48592\"},{\"content\":{\"connectorIds\":[],\"side\":\"TOP\"},\"type\":\"ConnectorPlacement.EquallySpacedRectSide\",\"uuid\":\"8005fa62-28e9-4165-9a4c-522b7a46ac73\"}]},\"type\":\"ConnectorPlacement.EquallySpacedConnector\",\"uuid\":\"9e1f4b76-5919-4e1e-b3b0-b0d66d2c7f29\"}],\"packageUris\":[\"http://schema.mathworks.com/mf0/Connector/R2020b\"],\"version\":\"1.0\"}"
  Power System Plant : Subsystem  VariantControl=Choice_1
      settings: PortSchema="{\"entries\":[{\"content\":{\"headerSize\":26,\"margin\":15,\"minimumSpacing\":25,\"sides\":[{\"content\":{\"connectorIds\":[\"In1\",\"In2\"]},\"type\":\"ConnectorPlacement.EquallySpacedRectSide\",\"uuid\":\"796081c6-2161-46d9-94c7-9250e1efb39a\"},{\"content\":{\"connectorIds\":[\"Out1\",\"Out2\"],\"side\":\"RIGHT\"},\"type\":\"ConnectorPlacement.EquallySpacedRectSide\",\"uuid\":\"b842dbfb-bf0a-4727-8e1c-eb47e2e48592\"},{\"content\":{\"connectorIds\":[],\"side\":\"TOP\"},\"type\":\"ConnectorPlacement.EquallySpacedRectSide\",\"uuid\":\"8005fa62-28e9-4165-9a4c-522b7a46ac73\"}]},\"type\":\"ConnectorPlacement.EquallySpacedConnector\",\"uuid\":\"9e1f4b76-5919-4e1e-b3b0-b0d66d2c7f29\"}],\"packageUris\":[\"http://schema.mathworks.com/mf0/Connector/R2020b\"],\"version\":\"1.0\"}"
  Bus Element Out1 : Outport  PortName=powerStates
  wires:
  Power System Control/1(actuatorCmd) -> Power System Plant/2(actuatorCmd)
  Power System Plant/2(sensorData) -> Power System Control/2(sensorData)
  Bus Element In1/1 -> Power System Control/1(attitudeStates)
  Power System Plant/1(powerStates) -> Bus Element Out1/1
  Bus Element In2/1 -> Power System Plant/1(attitudeStates)

== system asbCubeSatArchModel/CubeSat Mission Enterprise/Space Segment/CubeSat/Propulsion ==

== system asbCubeSatArchModel/CubeSat Mission Enterprise/Space Segment/CubeSat/Structures ==

== system asbCubeSatArchModel/CubeSat Mission Enterprise/Space Segment/CubeSat/Thermal ==

== system asbCubeSatArchModel/CubeSat Mission Enterprise/Space Segment/CubeSat/CDHS/Data Concentrator ==

== system asbCubeSatArchModel/CubeSat Mission Enterprise/Space Segment/CubeSat/CDHS/OnBoard Computer ==

== system asbCubeSatArchModel/CubeSat Mission Enterprise/Space Segment/CubeSat/Communications/Antenna ==

== system asbCubeSatArchModel/CubeSat Mission Enterprise/Space Segment/CubeSat/Communications/Tranceiver ==

== system asbCubeSatArchModel/CubeSat Mission Enterprise/Space Segment/CubeSat/GNC/Adapter ==
  In Bus Element : Inport  PortName=Environment
  Out Bus Element : Outport  PortName=Out
  wires:
  In Bus Element/1 -> Out Bus Element/1

== system asbCubeSatArchModel/CubeSat Mission Enterprise/Space Segment/CubeSat/GNC/Adapter1 ==
  In Bus Element : Inport  PortName=SensorsOut
  Out Bus Element : Outport  PortName=Input
  wires:
  In Bus Element/1 -> Out Bus Element/1

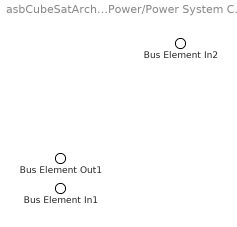
== system asbCubeSatArchModel/CubeSat Mission Enterprise/Space Segment/CubeSat/Power/Power System Control ==
  Bus Element In2 : Inport  PortName=attitudeStates
  Bus Element In1 : Inport  Port=2  PortName=sensorData
  Bus Element Out1 : Outport  PortName=actuatorCmd

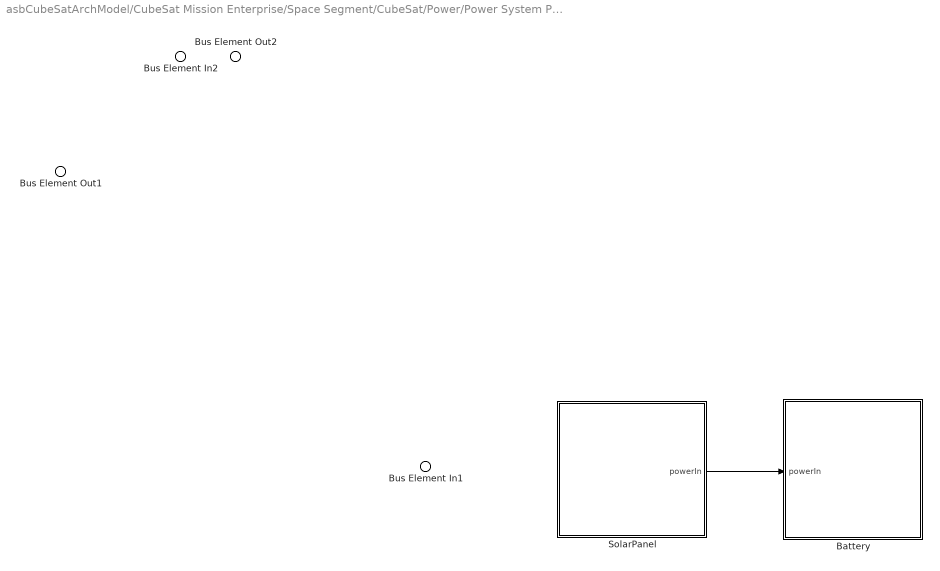
== system asbCubeSatArchModel/CubeSat Mission Enterprise/Space Segment/CubeSat/Power/Power System Plant ==
  Bus Element In2 : Inport  PortName=attitudeStates
  Bus Element In1 : Inport  Port=2  PortName=actuatorCmd
  Battery : Subsystem
      settings: PortSchema="{\"entries\":[{\"content\":{\"headerSize\":26,\"margin\":15,\"minimumSpacing\":25,\"sides\":[{\"content\":{\"connectorIds\":[\"In1\"]},\"type\":\"ConnectorPlacement.EquallySpacedRectSide\",\"uuid\":\"99007498-99ba-4c23-a0a0-87e1543943ee\"},{\"content\":{\"connectorIds\":[],\"side\":\"RIGHT\"},\"type\":\"ConnectorPlacement.EquallySpacedRectSide\",\"uuid\":\"554f3d31-4e95-4b23-9d3b-85f383ee0045\"},{\"content\":{\"connectorIds\":[],\"side\":\"TOP\"},\"type\":\"ConnectorPlacement.EquallySpacedRectSide\",\"uuid\":\"16cf11e7-d1a7-4edd-b8c5-05af2e73c5bd\"}]},\"type\":\"ConnectorPlacement.EquallySpacedConnector\",\"uuid\":\"0a651afa-d7fb-4b32-a21c-81d6f3c917ae\"}],\"packageUris\":[\"http://schema.mathworks.com/mf0/Connector/R2020b\"],\"version\":\"1.0\"}"
  SolarPanel : Subsystem  RequirementInfo="{}  %GIDa_4f725f0c_e8f4_4f8d_a212_700d35e9a783"
      settings: PortSchema="{\"entries\":[{\"content\":{\"headerSize\":26,\"margin\":15,\"minimumSpacing\":25,\"sides\":[{\"content\":{\"connectorIds\":[]},\"type\":\"ConnectorPlacement.EquallySpacedRectSide\",\"uuid\":\"bdb7f036-cfc5-488a-888f-b9d18995973e\"},{\"content\":{\"connectorIds\":[\"Out1\"],\"side\":\"RIGHT\"},\"type\":\"ConnectorPlacement.EquallySpacedRectSide\",\"uuid\":\"bf580f20-7193-4743-ad48-17eb92535429\"},{\"content\":{\"connectorIds\":[],\"side\":\"TOP\"},\"type\":\"ConnectorPlacement.EquallySpacedRectSide\",\"uuid\":\"da6f3a46-474d-4698-8115-df2cb74be4ae\"}]},\"type\":\"ConnectorPlacement.EquallySpacedConnector\",\"uuid\":\"514a736b-bd6f-43cb-ac87-4eaa6b5005de\"}],\"packageUris\":[\"http://schema.mathworks.com/mf0/Connector/R2020b\"],\"version\":\"1.0\"}"
  Bus Element Out2 : Outport  PortName=powerStates
  Bus Element Out1 : Outport  Port=2  PortName=sensorData
  wires:
  SolarPanel/1(powerIn) -> Battery/1(powerIn)

== system asbCubeSatArchModel/CubeSat Mission Enterprise/Space Segment/CubeSat/Power/Power System Plant/Battery ==
  Bus Element In1 : Inport  PortName=powerIn
  BatteryCell : Subsystem
      settings: PortSchema="{\"entries\":[{\"content\":{\"headerSize\":26,\"margin\":15,\"minimumSpacing\":25,\"sides\":[{\"content\":{\"connectorIds\":[]},\"type\":\"ConnectorPlacement.EquallySpacedRectSide\",\"uuid\":\"bdb7f036-cfc5-488a-888f-b9d18995973e\"},{\"content\":{\"connectorIds\":[],\"side\":\"RIGHT\"},\"type\":\"ConnectorPlacement.EquallySpacedRectSide\",\"uuid\":\"bf580f20-7193-4743-ad48-17eb92535429\"},{\"content\":{\"connectorIds\":[],\"side\":\"TOP\"},\"type\":\"ConnectorPlacement.EquallySpacedRectSide\",\"uuid\":\"da6f3a46-474d-4698-8115-df2cb74be4ae\"}]},\"type\":\"ConnectorPlacement.EquallySpacedConnector\",\"uuid\":\"514a736b-bd6f-43cb-ac87-4eaa6b5005de\"}],\"packageUris\":[\"http://schema.mathworks.com/mf0/Connector/19700101\"],\"version\":\"1.0\"}"

== system asbCubeSatArchModel/CubeSat Mission Enterprise/Space Segment/CubeSat/Power/Power System Plant/SolarPanel ==
  SolarPanelCell : Subsystem
      settings: PortSchema="{\"entries\":[{\"content\":{\"headerSize\":26,\"margin\":15,\"minimumSpacing\":25,\"sides\":[{\"content\":{\"connectorIds\":[]},\"type\":\"ConnectorPlacement.EquallySpacedRectSide\",\"uuid\":\"bdb7f036-cfc5-488a-888f-b9d18995973e\"},{\"content\":{\"connectorIds\":[],\"side\":\"RIGHT\"},\"type\":\"ConnectorPlacement.EquallySpacedRectSide\",\"uuid\":\"bf580f20-7193-4743-ad48-17eb92535429\"},{\"content\":{\"connectorIds\":[],\"side\":\"TOP\"},\"type\":\"ConnectorPlacement.EquallySpacedRectSide\",\"uuid\":\"da6f3a46-474d-4698-8115-df2cb74be4ae\"}]},\"type\":\"ConnectorPlacement.EquallySpacedConnector\",\"uuid\":\"514a736b-bd6f-43cb-ac87-4eaa6b5005de\"}],\"packageUris\":[\"http://schema.mathworks.com/mf0/Connector/19700101\"],\"version\":\"1.0\"}"
  Bus Element Out1 : Outport  PortName=powerIn

== system asbCubeSatArchModel/CubeSat Mission Enterprise/Space Segment/CubeSat/Power/Power System Plant/Battery/BatteryCell ==

== system asbCubeSatArchModel/CubeSat Mission Enterprise/Space Segment/CubeSat/Power/Power System Plant/SolarPanel/SolarPanelCell ==
